simulink model "ex3s"  (R2022a)
settings: Solver=VariableStepAuto  StartTime=0.0  StopTime=10.0  RelTol=1e-3
settings Model: Creator=giova  LastModifiedBy=giova

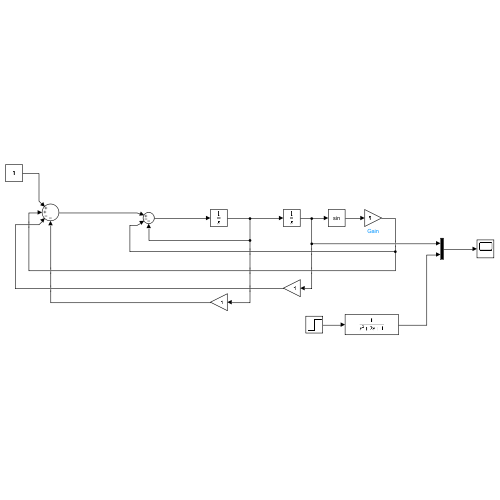
[thumbnail: Simulink's stored preview of the top-level diagram]
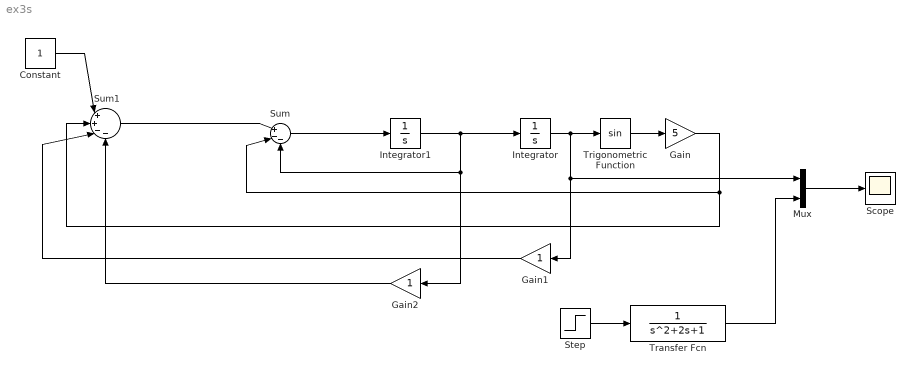
== system ex3s ==
  Constant : Constant
  Gain : Gain  Gain=5
  Gain1 : Gain
  Gain2 : Gain
  Integrator : Integrator
  Integrator1 : Integrator
  Mux : Mux  Inputs=2
  Scope : Scope
  Step : Step  SampleTime=0
  Sum : Sum  Inputs=|+--
  Sum1 : Sum  Inputs=|++--
  Transfer Fcn : TransferFcn
  Trigonometric Function : Trigonometry
  wires:
  Sum/1 -> Integrator1/1
  Integrator1/1 -> Gain2/1, Sum/3, Integrator/1
  Integrator/1 -> Mux/1, Gain1/1, Trigonometric Function/1
  Trigonometric Function/1 -> Gain/1
  Gain/1 -> Sum1/2, Sum/2
  Sum1/1 -> Sum/1
  Constant/1 -> Sum1/1
  Gain1/1 -> Sum1/3
  Gain2/1 -> Sum1/4
  Step/1 -> Transfer Fcn/1
  Transfer Fcn/1 -> Mux/2
  Mux/1 -> Scope/1
